simulink model "fw_io_out_sim"  (R2026b)
settings: Solver=VariableStepAuto
undefined symbols (not defined in the file or in its folder): Ts
settings Model: Creator=aomar  LastModifiedBy=aomar

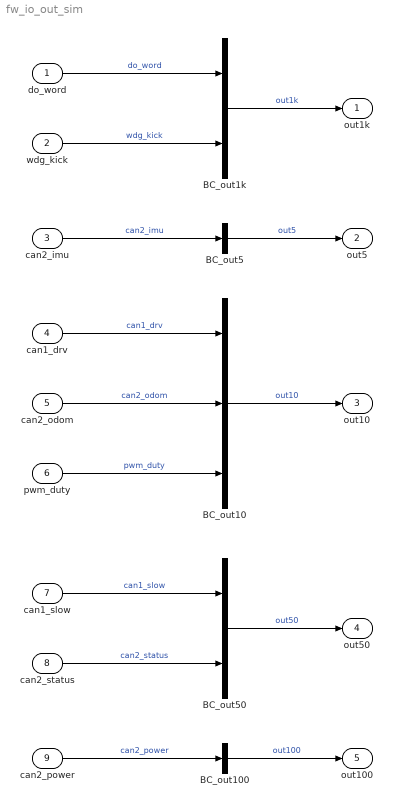
== system fw_io_out_sim ==
  do_word : Inport  OutDataTypeStr=uint32  SampleTime=Ts.base
  wdg_kick : Inport  Port=2  OutDataTypeStr=boolean  SampleTime=Ts.base
  can2_imu : Inport  Port=3  OutDataTypeStr=Bus: Bus_CanFrame64  SampleTime=Ts.imu
  can1_drv : Inport  Port=4  OutDataTypeStr=Bus: Bus_Can1_McuFast  SampleTime=Ts.ctrl
  can2_odom : Inport  Port=5  OutDataTypeStr=Bus: Bus_CanFrame64  SampleTime=Ts.ctrl
  pwm_duty : Inport  Port=6  OutDataTypeStr=single  PortDimensions=4  SampleTime=Ts.ctrl
  can1_slow : Inport  Port=7  OutDataTypeStr=Bus: Bus_Can1_McuSlow  SampleTime=Ts.comm
  can2_status : Inport  Port=8  OutDataTypeStr=Bus: Bus_CanFrame64  SampleTime=Ts.comm
  can2_power : Inport  Port=9  OutDataTypeStr=Bus: Bus_CanFrame64  SampleTime=Ts.hk
  BC_out10 : BusCreator  Inputs=3  OutDataTypeStr=Bus: Bus_McuOut10  NonVirtualBus=on
      settings: InheritFromInputs=off
  BC_out100 : BusCreator  Inputs=1  OutDataTypeStr=Bus: Bus_McuOut100  NonVirtualBus=on
      settings: InheritFromInputs=off
  BC_out1k : BusCreator  Inputs=2  OutDataTypeStr=Bus: Bus_McuOut1k  NonVirtualBus=on
      settings: InheritFromInputs=off
  BC_out5 : BusCreator  Inputs=1  OutDataTypeStr=Bus: Bus_McuOut5  NonVirtualBus=on
      settings: InheritFromInputs=off
  BC_out50 : BusCreator  Inputs=2  OutDataTypeStr=Bus: Bus_McuOut50  NonVirtualBus=on
      settings: InheritFromInputs=off
  out1k : Outport  OutDataTypeStr=Bus: Bus_McuOut1k
  out5 : Outport  Port=2  OutDataTypeStr=Bus: Bus_McuOut5
  out10 : Outport  Port=3  OutDataTypeStr=Bus: Bus_McuOut10
  out50 : Outport  Port=4  OutDataTypeStr=Bus: Bus_McuOut50
  out100 : Outport  Port=5  OutDataTypeStr=Bus: Bus_McuOut100
  wires:
  do_word/1 -> BC_out1k/1  "do_word"
  wdg_kick/1 -> BC_out1k/2  "wdg_kick"
  can2_imu/1 -> BC_out5/1  "can2_imu"
  can1_drv/1 -> BC_out10/1  "can1_drv"
  can2_odom/1 -> BC_out10/2  "can2_odom"
  pwm_duty/1 -> BC_out10/3  "pwm_duty"
  can1_slow/1 -> BC_out50/1  "can1_slow"
  can2_status/1 -> BC_out50/2  "can2_status"
  can2_power/1 -> BC_out100/1  "can2_power"
  BC_out1k/1 -> out1k/1  "out1k"
  BC_out5/1 -> out5/1  "out5"
  BC_out10/1 -> out10/1  "out10"
  BC_out50/1 -> out50/1  "out50"
  BC_out100/1 -> out100/1  "out100"
